simulink model "system_model_backup"  (R2025b)
settings: Solver=ode45  StartTime=0.0  StopTime=2  MaxStep=0.001  RelTol=1e-3
undefined symbols (not defined in the file): p
settings Model: Creator=Dawid  LastModifiedBy=Dawid

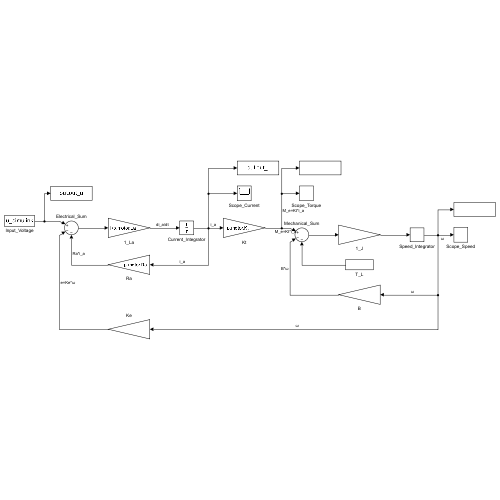
[thumbnail: Simulink's stored preview of the top-level diagram]
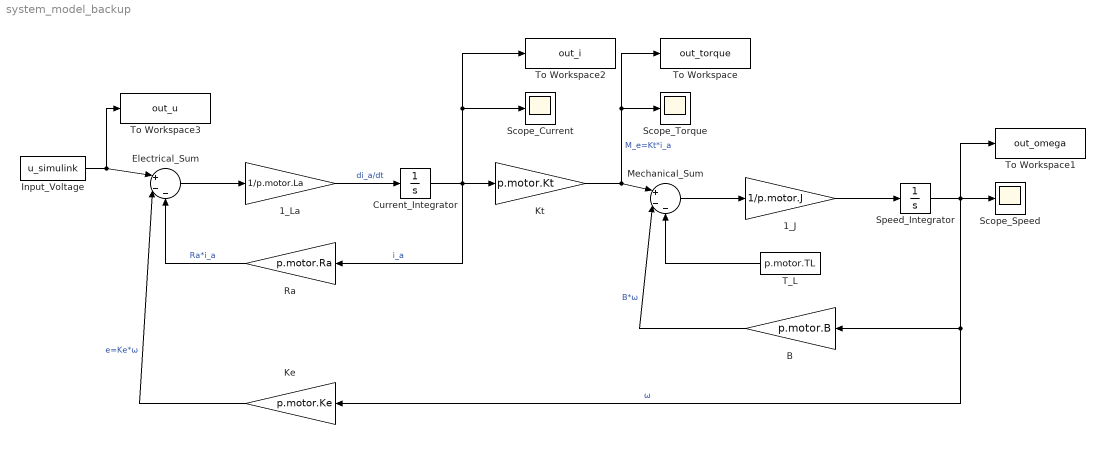
== system system_model_backup ==
  1_J : Gain  Gain=1/p.motor.J
  1_La : Gain  Gain=1/p.motor.La
  B : Gain  Gain=p.motor.B
  Current_Integrator : Integrator  InitialCondition=p.initial.i_a
  Electrical_Sum : Sum  Inputs=|+--
  Input_Voltage : FromWorkspace  VariableName=u_simulink  Interpolate=off  OutputAfterFinalValue=Holding final value
  Ke : Gain  Gain=p.motor.Ke
  Kt : Gain  Gain=p.motor.Kt
  Mechanical_Sum : Sum  Inputs=|+--
  Ra : Gain  Gain=p.motor.Ra
  Scope_Current : Scope
      settings: ActiveDisplayYMinimum=-0.43190634429427927  ActiveDisplayYMaximum=3.8871570986485144
  Scope_Speed : Scope
      settings: ActiveDisplayYMinimum=-1.3020216523409809  ActiveDisplayYMaximum=11.71819487106883  DataLoggingVariableName=ScopeData2
  Scope_Torque : Scope
      settings: ActiveDisplayYMinimum=-0.21595317214713963  ActiveDisplayYMaximum=1.9435785493242572
  Speed_Integrator : Integrator  InitialCondition=p.initial.omega
  T_L : Constant  Value=p.motor.TL
  To Workspace : ToWorkspace  VariableName=out_torque  SaveFormat=Timeseries  SampleTime=-1
  To Workspace1 : ToWorkspace  VariableName=out_omega  SaveFormat=Timeseries  SampleTime=-1
  To Workspace2 : ToWorkspace  VariableName=out_i  SaveFormat=Timeseries  SampleTime=-1
  To Workspace3 : ToWorkspace  VariableName=out_u  SaveFormat=Timeseries  SampleTime=-1
  wires:
  Input_Voltage/1 -> To Workspace3/1, Electrical_Sum/1
  Electrical_Sum/1 -> 1_La/1
  1_La/1 -> Current_Integrator/1  "di_a/dt"
  Current_Integrator/1 -> Scope_Current/1, To Workspace2/1, Kt/1, Ra/1  "i_a"
  Ra/1 -> Electrical_Sum/3  "Ra*i_a"
  Kt/1 -> Scope_Torque/1, To Workspace/1, Mechanical_Sum/1  "M_e=Kt*i_a"
  T_L/1 -> Mechanical_Sum/3
  Mechanical_Sum/1 -> 1_J/1
  1_J/1 -> Speed_Integrator/1
  Speed_Integrator/1 -> To Workspace1/1, Scope_Speed/1, B/1, Ke/1  "ω"
  B/1 -> Mechanical_Sum/2  "B*ω"
  Ke/1 -> Electrical_Sum/2  "e=Ke*ω"
